simulink model "single_phase_pll_analysis"  (R2026b)
settings: Solver=ode1  StopTime=param.sim.simlength  FixedStep=param.glb_time.ts_inv
values from neighbouring files (symbols this model uses):
  param = struct()    [init_model.m]    (also in plotting_results_plls.m = evalin('base', 'param'); run_test_cases.m = param0)
undefined symbols (not defined in the file or in its folder): magnitude
libraries: discrete_time_low_pass_filter x6
settings Model: Creator=dbagn  LastModifiedBy=dbagn
settings DataIOCC: DSMLogging=off  ReturnWorkspaceOutputs=off  SaveOutput=off  SaveTime=off  SignalLogging=off
settings SimscapeCC: SimscapeUseEnergyAccounting=off

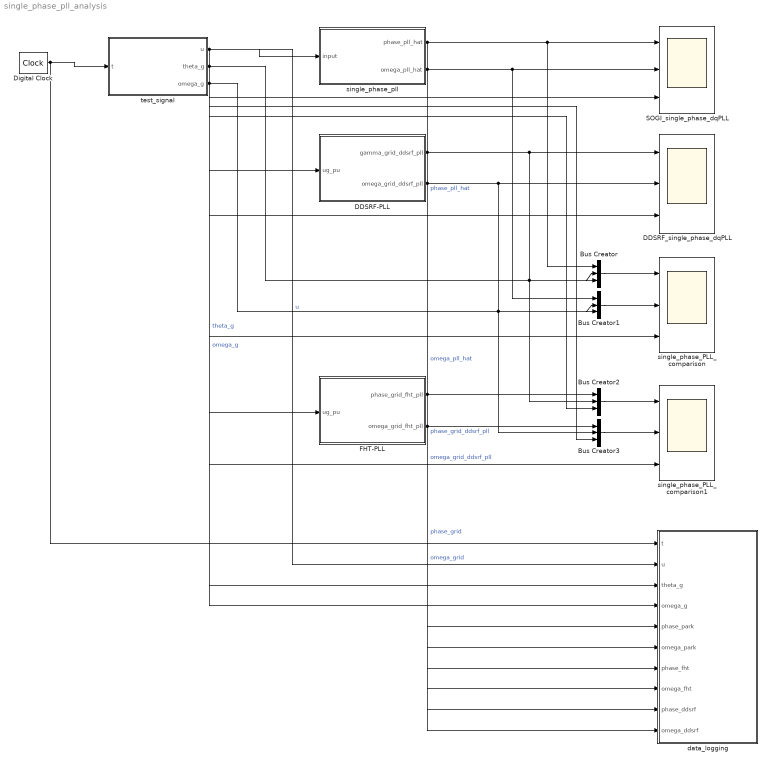
== system single_phase_pll_analysis ==
  Bus Creator{,1..3} (4 alike) : BusCreator  Inputs=3
  DDSRF-PLL : Subsystem
  DDSRF_single_phase_dqPLL : Scope  NumInputPorts=3
      settings: ActiveDisplayYMinimum=-3.9119372895053015  ActiveDisplayYMaximum=3.9180108973262389
  Digital Clock : DigitalClock  SampleTime=param.glb_time.ts_inv
  FHT-PLL : Subsystem
  SOGI_single_phase_dqPLL : Scope  NumInputPorts=3
      settings: ActiveDisplayYMinimum=-3.9194465033742367  ActiveDisplayYMaximum=3.9240760802470063  DataLoggingVariableName=ScopeData2
  data_logging : Subsystem
  single_phase_PLL_comparison : Scope  NumInputPorts=3
      settings: ActiveDisplayYMinimum=-3.9263229152471837  ActiveDisplayYMaximum=3.9266269550757258  DataLoggingVariableName=ScopeData3
  single_phase_PLL_comparison1 : Scope  NumInputPorts=3
      settings: ActiveDisplayYMinimum=-3.9176213284578751  ActiveDisplayYMaximum=3.9220307130849243  DataLoggingVariableName=ScopeData4
  single_phase_pll : Subsystem
  test_signal : MATLAB Function  TreatAsAtomicUnit=on  mask(test_signal){p=param.test}
      mask prompts: p "test signal (param.test)"
      mask help: Single-phase test voltage in pu of the nominal peak, angle theta_g and pulsation omega_g [pu] of its fundamental. p: struct of private/test_param.m (param.test).
  wires:
  DDSRF-PLL/1(gamma_grid_ddsrf_pll) -> Bus Creator2/2, Bus Creator/2, DDSRF_single_phase_dqPLL/1, data_logging/9(phase_ddsrf)  "phase_grid_ddsrf_pll"
  DDSRF-PLL/2(omega_grid_ddsrf_pll) -> Bus Creator3/2, Bus Creator1/2, DDSRF_single_phase_dqPLL/2, data_logging/10(omega_ddsrf)  "omega_grid_ddsrf_pll"
  single_phase_pll/1(phase_pll_hat) -> SOGI_single_phase_dqPLL/1, Bus Creator/1, data_logging/5(phase_park)  "phase_pll_hat"
  single_phase_pll/2(omega_pll_hat) -> Bus Creator1/1, SOGI_single_phase_dqPLL/2, data_logging/6(omega_park)  "omega_pll_hat"
  Bus Creator/1 -> single_phase_PLL_comparison/1
  Bus Creator1/1 -> single_phase_PLL_comparison/2
  Bus Creator3/1 -> single_phase_PLL_comparison1/2
  Bus Creator2/1 -> single_phase_PLL_comparison1/1
  FHT-PLL/1(phase_grid_fht_pll) -> Bus Creator2/1, data_logging/7(phase_fht)  "phase_grid"
  FHT-PLL/2(omega_grid_fht_pll) -> Bus Creator3/1, data_logging/8(omega_fht)  "omega_grid"
  Digital Clock/1 -> test_signal/1(t), data_logging/1(t)
  test_signal/1(u) -> single_phase_pll/1(input), DDSRF-PLL/1(ug_pu), FHT-PLL/1(ug_pu), SOGI_single_phase_dqPLL/3, DDSRF_single_phase_dqPLL/3, single_phase_PLL_comparison/3, single_phase_PLL_comparison1/3, data_logging/2(u)  "u"
  test_signal/2(theta_g) -> Bus Creator/3, Bus Creator2/3, data_logging/3(theta_g)  "theta_g"
  test_signal/3(omega_g) -> Bus Creator1/3, Bus Creator3/3, data_logging/4(omega_g)  "omega_g"

== system single_phase_pll_analysis/DDSRF-PLL ==
  ug_pu : Inport
  Goto Tag Visibility : GotoTagVisibility  GotoTag=Vgrid_unorm_ddsrf
  pll_stageA : Subsystem
  pll_stageB : Subsystem
  gamma_grid_ddsrf_pll : Outport
  omega_grid_ddsrf_pll : Outport  Port=2
  wires:
  pll_stageB/1(phase_grid_ddsrf_pll) -> pll_stageA/1(gamma_grid), gamma_grid_ddsrf_pll/1
  pll_stageA/2(u_grid_pos_eta) -> pll_stageB/2(u_grid_pos_eta)  "u_grid_pos_eta"
  pll_stageA/1(u_grid_pos_xi) -> pll_stageB/1(u_grid_pos_xi)  "u_grid_pos_xi"
  pll_stageB/2(omega_grid_ddsrf_pll) -> omega_grid_ddsrf_pll/1
  ug_pu/1 -> pll_stageA/2(ug_pu)

== system single_phase_pll_analysis/FHT-PLL ==
  ug_pu : Inport
  Goto Tag Visibility : GotoTagVisibility  GotoTag=Vgrid_unorm_fht
  pll_stageA : Subsystem
  pll_stageB : Subsystem
  phase_grid_fht_pll : Outport
  omega_grid_fht_pll : Outport  Port=2
  wires:
  pll_stageB/2(omega_grid_ddsrf_pll) -> omega_grid_fht_pll/1
  pll_stageA/1(u_grid_xi) -> pll_stageB/1(u_grid_pos_xi)  "u_grid_pos_xi"
  pll_stageA/2(u_grid_eta) -> pll_stageB/2(u_grid_pos_eta)  "u_grid_pos_eta"
  pll_stageB/1(phase_grid_ddsrf_pll) -> phase_grid_fht_pll/1, pll_stageA/1(gamma_grid)
  ug_pu/1 -> pll_stageA/2(ug_pu)

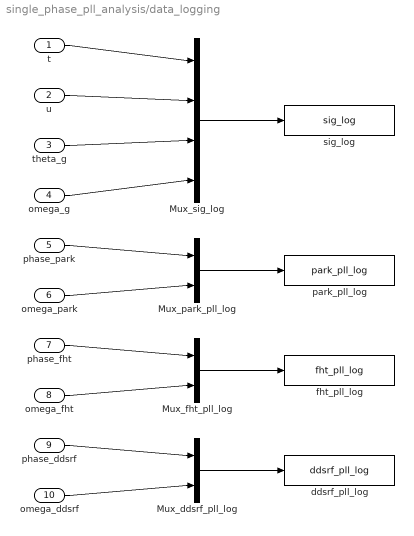
== system single_phase_pll_analysis/data_logging ==
  t : Inport
  u : Inport  Port=2
  theta_g : Inport  Port=3
  omega_g : Inport  Port=4
  phase_park : Inport  Port=5
  omega_park : Inport  Port=6
  phase_fht : Inport  Port=7
  omega_fht : Inport  Port=8
  phase_ddsrf : Inport  Port=9
  omega_ddsrf : Inport  Port=10
  Mux_ddsrf_pll_log : Mux  Inputs=2
  Mux_fht_pll_log : Mux  Inputs=2
  Mux_park_pll_log : Mux  Inputs=2
  Mux_sig_log : Mux
  ddsrf_pll_log : ToWorkspace  VariableName=ddsrf_pll_log  SampleTime=-1
      settings: MaxDataPoints=param.glb_time.Ns_afe
  fht_pll_log : ToWorkspace  VariableName=fht_pll_log  SampleTime=-1
      settings: MaxDataPoints=param.glb_time.Ns_afe
  park_pll_log : ToWorkspace  VariableName=park_pll_log  SampleTime=-1
      settings: MaxDataPoints=param.glb_time.Ns_afe
  sig_log : ToWorkspace  VariableName=sig_log  SampleTime=-1
      settings: MaxDataPoints=param.glb_time.Ns_afe
  wires:
  t/1 -> Mux_sig_log/1
  u/1 -> Mux_sig_log/2
  theta_g/1 -> Mux_sig_log/3
  omega_g/1 -> Mux_sig_log/4
  Mux_sig_log/1 -> sig_log/1
  phase_park/1 -> Mux_park_pll_log/1
  omega_park/1 -> Mux_park_pll_log/2
  Mux_park_pll_log/1 -> park_pll_log/1
  phase_fht/1 -> Mux_fht_pll_log/1
  omega_fht/1 -> Mux_fht_pll_log/2
  Mux_fht_pll_log/1 -> fht_pll_log/1
  phase_ddsrf/1 -> Mux_ddsrf_pll_log/1
  omega_ddsrf/1 -> Mux_ddsrf_pll_log/2
  Mux_ddsrf_pll_log/1 -> ddsrf_pll_log/1

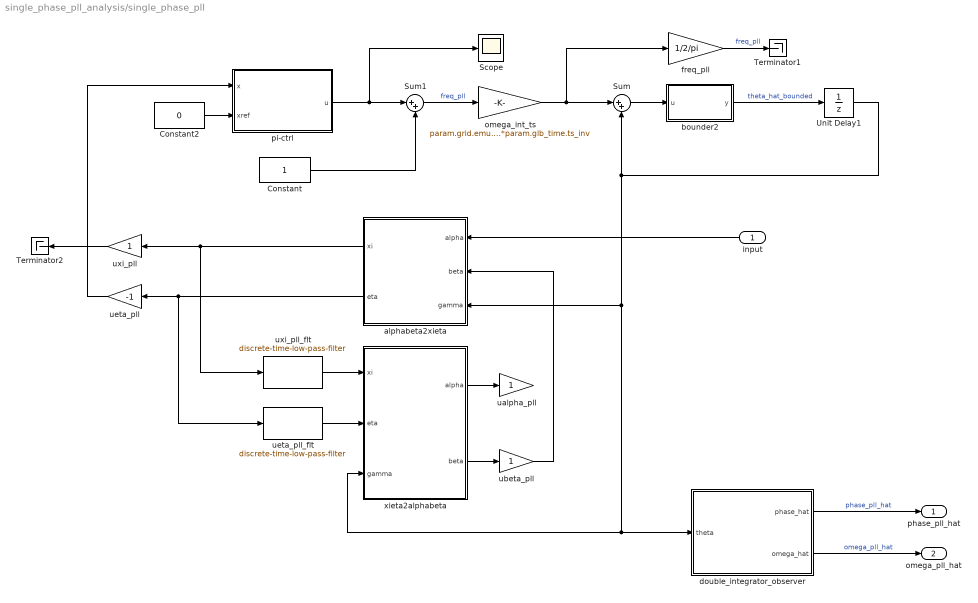
== system single_phase_pll_analysis/single_phase_pll ==
  input : Inport
  Constant : Constant
  Constant2 : Constant  Value=0
  Scope : Scope
      settings: ActiveDisplayYMinimum=-1.1813345026503461  ActiveDisplayYMaximum=0.50653477204197639
  Sum : Sum  Inputs=|++
  Sum1 : Sum  Inputs=|++
  Terminator1 : Terminator
  Terminator2 : Terminator
  Unit Delay1 : UnitDelay  SampleTime=-1
  alphabeta2xieta : MATLAB Function  TreatAsAtomicUnit=on
  bounder2 : MATLAB Function  TreatAsAtomicUnit=on
  double_integrator_observer : Subsystem
  freq_pll : Gain  Gain=1/2/pi
  omega_int_ts : Gain  Gain=param.grid.emu.omega_grid_nom*param.glb_time.ts_inv
  pi-ctrl : Subsystem  mask{kp=param.afe.pll.park.kp, ki=param.afe.pll.park.ki, ts=param.glb_time.ts_inv, sat_pos=param.afe.pll.park.sat_pos, sat_neg=param.afe.pll.park.sat_neg}
  ualpha_pll : Gain
  ubeta_pll : Gain
  ueta_pll : Gain  Gain=-1
  ueta_pll_flt : discrete_time_low_pass_filter/discrete-time-low-pass-filter  tau=param.afe.pll.park.tau  ts=param.glb_time.ts_inv
  uxi_pll : Gain
  uxi_pll_flt : discrete_time_low_pass_filter/discrete-time-low-pass-filter  tau=param.afe.pll.park.tau  ts=param.glb_time.ts_inv
  xieta2alphabeta : MATLAB Function  TreatAsAtomicUnit=on
  phase_pll_hat : Outport
  omega_pll_hat : Outport  Port=2
  wires:
  Sum/1 -> bounder2/1(u)
  alphabeta2xieta/1(xi) -> uxi_pll/1, uxi_pll_flt/1
  xieta2alphabeta/2(beta) -> ubeta_pll/1
  alphabeta2xieta/2(eta) -> ueta_pll/1, ueta_pll_flt/1
  omega_int_ts/1 -> freq_pll/1, Sum/1
  double_integrator_observer/1(phase_hat) -> phase_pll_hat/1  "phase_pll_hat"
  input/1 -> alphabeta2xieta/1(alpha)
  freq_pll/1 -> Terminator1/1  "freq_pll"
  ueta_pll_flt/1 -> xieta2alphabeta/2(eta)
  uxi_pll_flt/1 -> xieta2alphabeta/1(xi)
  ueta_pll/1 -> pi-ctrl/1(x)
  Sum1/1 -> omega_int_ts/1  "freq_pll"
  Constant2/1 -> pi-ctrl/2(xref)
  uxi_pll/1 -> Terminator2/1
  ubeta_pll/1 -> alphabeta2xieta/2(beta)
  xieta2alphabeta/1(alpha) -> ualpha_pll/1
  pi-ctrl/1(u) -> Sum1/1, Scope/1
  Constant/1 -> Sum1/2
  Unit Delay1/1 -> Sum/2, alphabeta2xieta/3(gamma), xieta2alphabeta/3(gamma), double_integrator_observer/1(theta)
  bounder2/1(y) -> Unit Delay1/1  "theta_hat_bounded"
  double_integrator_observer/2(omega_hat) -> omega_pll_hat/1  "omega_pll_hat"

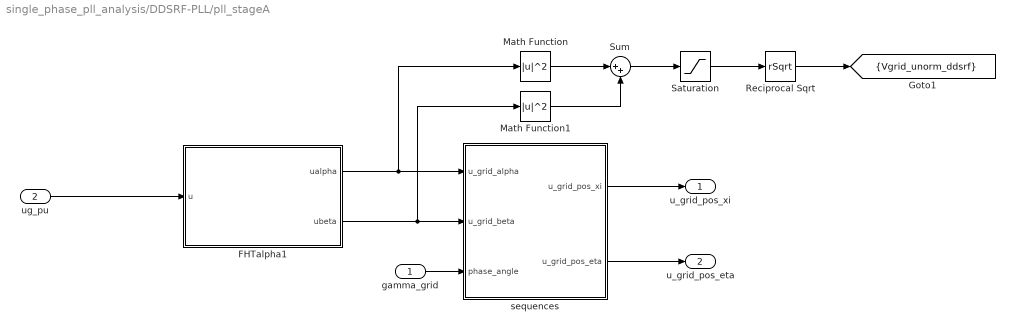
== system single_phase_pll_analysis/DDSRF-PLL/pll_stageA ==
  gamma_grid : Inport
  ug_pu : Inport  Port=2
  FHTalpha1 : Subsystem
  Math Function : Math  Operator=magnitude^2  SignedPower=on
  Math Function1 : Math  Operator=magnitude^2  SignedPower=on
  Reciprocal Sqrt : Sqrt  Operator=rSqrt
  Saturation : Saturate  UpperLimit=inf  LowerLimit=0.02
  Sum : Sum  Inputs=|++
  sequences : Subsystem
  u_grid_pos_xi : Outport  VectorParamsAs1DForOutWhenUnconnected=off
  u_grid_pos_eta : Outport  Port=2  VectorParamsAs1DForOutWhenUnconnected=off
  tag scope: Vgrid_unorm_ddsrf=scoped
  wires:
  Saturation/1 -> Reciprocal Sqrt/1
  Reciprocal Sqrt/1 -> [Vgrid_unorm_ddsrf]
  Sum/1 -> Saturation/1
  Math Function1/1 -> Sum/2
  Math Function/1 -> Sum/1
  FHTalpha1/2(ubeta) -> Math Function1/1, sequences/2(u_grid_beta)
  FHTalpha1/1(ualpha) -> Math Function/1, sequences/1(u_grid_alpha)
  sequences/1(u_grid_pos_xi) -> u_grid_pos_xi/1
  sequences/2(u_grid_pos_eta) -> u_grid_pos_eta/1
  gamma_grid/1 -> sequences/3(phase_angle)
  ug_pu/1 -> FHTalpha1/1(u)

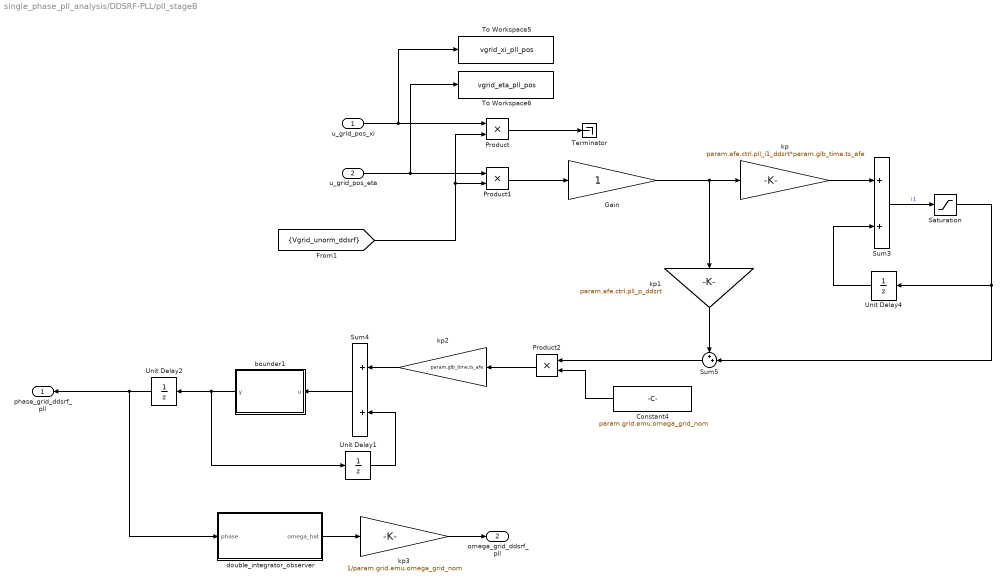
== system single_phase_pll_analysis/DDSRF-PLL/pll_stageB ==
  u_grid_pos_xi : Inport
  u_grid_pos_eta : Inport  Port=2
  Constant4 : Constant  Value=param.grid.emu.omega_grid_nom
  Gain : Gain
  Product : Product  RndMeth=Zero
  Product1 : Product  RndMeth=Zero
  Product2 : Product  RndMeth=Zero
  Saturation : Saturate  UpperLimit=1.5  LowerLimit=0.5
  Sum3 : Sum  SaturateOnIntegerOverflow=on
  Sum4 : Sum  SaturateOnIntegerOverflow=on
  Sum5 : Sum  Inputs=++|
  Terminator : Terminator
  To Workspace5 : ToWorkspace  VariableName=vgrid_xi_pll_pos  SampleTime=-1
      settings: MaxDataPoints=param.glb_time.Ns_afe
  To Workspace6 : ToWorkspace  VariableName=vgrid_eta_pll_pos  SampleTime=-1
      settings: MaxDataPoints=param.glb_time.Ns_afe
  Unit Delay1 : UnitDelay  SampleTime=-1
  Unit Delay2 : UnitDelay  SampleTime=-1
  Unit Delay4 : UnitDelay  SampleTime=-1
  bounder1 : MATLAB Function  TreatAsAtomicUnit=on
  double_integrator_observer : Subsystem
  kp : Gain  Gain=param.afe.ctrl.pll_i1_ddsrt*param.glb_time.ts_afe  SaturateOnIntegerOverflow=on  OutDataTypeStr=Inherit: Same as input  ParamDataTypeStr=Inherit: Same as input
  kp1 : Gain  Gain=param.afe.ctrl.pll_p_ddsrt  SaturateOnIntegerOverflow=on  OutDataTypeStr=Inherit: Same as input  ParamDataTypeStr=Inherit: Same as input
  kp2 : Gain  Gain=param.glb_time.ts_afe  SaturateOnIntegerOverflow=on  OutDataTypeStr=Inherit: Same as input  ParamDataTypeStr=Inherit: Same as input
  kp3 : Gain  Gain=1/param.grid.emu.omega_grid_nom  SaturateOnIntegerOverflow=on  OutDataTypeStr=Inherit: Same as input  ParamDataTypeStr=Inherit: Same as input
  phase_grid_ddsrf_pll : Outport  VectorParamsAs1DForOutWhenUnconnected=off
  omega_grid_ddsrf_pll : Outport  Port=2  VectorParamsAs1DForOutWhenUnconnected=off
  wires:
  Unit Delay2/1 -> double_integrator_observer/1(phase), phase_grid_ddsrf_pll/1
  kp1/1 -> Sum5/1
  Product2/1 -> kp2/1
  u_grid_pos_eta/1 -> Product1/1, To Workspace6/1
  u_grid_pos_xi/1 -> To Workspace5/1, Product/1
  bounder1/1(y) -> Unit Delay1/1, Unit Delay2/1
  Sum5/1 -> Product2/1
  kp/1 -> Sum3/1
  [Vgrid_unorm_ddsrf] -> Product1/2, Product/2
  Constant4/1 -> Product2/2
  kp2/1 -> Sum4/1
  Sum3/1 -> Saturation/1  "i1"
  Unit Delay1/1 -> Sum4/2
  Sum4/1 -> bounder1/1(u)
  Unit Delay4/1 -> Sum3/2
  double_integrator_observer/1(omega_hat) -> kp3/1
  Product/1 -> Terminator/1
  kp3/1 -> omega_grid_ddsrf_pll/1
  Product1/1 -> Gain/1
  Gain/1 -> kp1/1, kp/1
  Saturation/1 -> Unit Delay4/1, Sum5/2

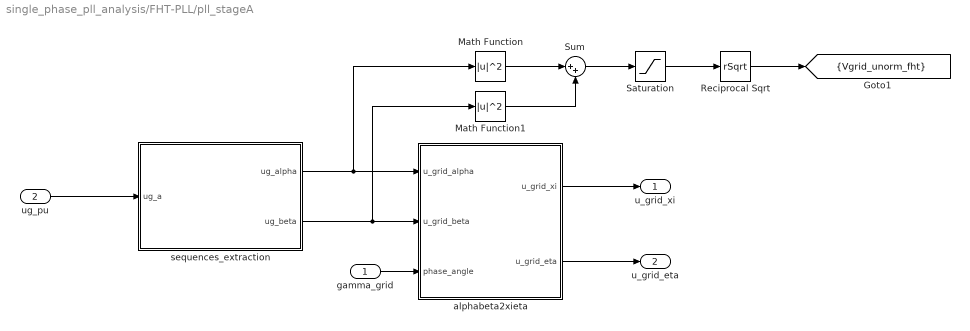
== system single_phase_pll_analysis/FHT-PLL/pll_stageA ==
  gamma_grid : Inport
  ug_pu : Inport  Port=2
  Math Function : Math  Operator=magnitude^2  SignedPower=on
  Math Function1 : Math  Operator=magnitude^2  SignedPower=on
  Reciprocal Sqrt : Sqrt  Operator=rSqrt
  Saturation : Saturate  UpperLimit=inf  LowerLimit=0.02
  Sum : Sum  Inputs=|++
  alphabeta2xieta : Subsystem
  sequences_extraction : Subsystem
  u_grid_xi : Outport  VectorParamsAs1DForOutWhenUnconnected=off
  u_grid_eta : Outport  Port=2  VectorParamsAs1DForOutWhenUnconnected=off
  tag scope: Vgrid_unorm_fht=scoped
  wires:
  gamma_grid/1 -> alphabeta2xieta/3(phase_angle)
  alphabeta2xieta/2(u_grid_eta) -> u_grid_eta/1
  alphabeta2xieta/1(u_grid_xi) -> u_grid_xi/1
  sequences_extraction/1(ug_alpha) -> Math Function/1, alphabeta2xieta/1(u_grid_alpha)
  sequences_extraction/2(ug_beta) -> Math Function1/1, alphabeta2xieta/2(u_grid_beta)
  Math Function/1 -> Sum/1
  Math Function1/1 -> Sum/2
  Sum/1 -> Saturation/1
  Reciprocal Sqrt/1 -> [Vgrid_unorm_fht]
  Saturation/1 -> Reciprocal Sqrt/1
  ug_pu/1 -> sequences_extraction/1(ug_a)

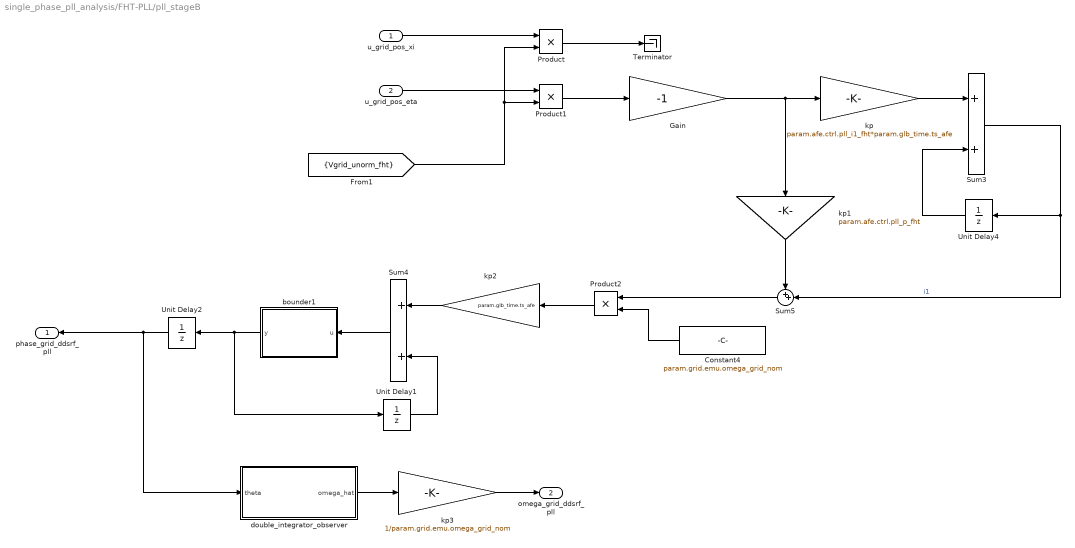
== system single_phase_pll_analysis/FHT-PLL/pll_stageB ==
  u_grid_pos_xi : Inport
  u_grid_pos_eta : Inport  Port=2
  Constant4 : Constant  Value=param.grid.emu.omega_grid_nom
  Gain : Gain  Gain=-1
  Product : Product  RndMeth=Zero
  Product1 : Product  RndMeth=Zero
  Product2 : Product  RndMeth=Zero
  Sum3 : Sum  SaturateOnIntegerOverflow=on
  Sum4 : Sum  SaturateOnIntegerOverflow=on
  Sum5 : Sum  Inputs=++|
  Terminator : Terminator
  Unit Delay1 : UnitDelay  SampleTime=-1
  Unit Delay2 : UnitDelay  SampleTime=-1
  Unit Delay4 : UnitDelay  SampleTime=-1
  bounder1 : MATLAB Function  TreatAsAtomicUnit=on
  double_integrator_observer : Subsystem
  kp : Gain  Gain=param.afe.ctrl.pll_i1_fht*param.glb_time.ts_afe  SaturateOnIntegerOverflow=on  OutDataTypeStr=Inherit: Same as input  ParamDataTypeStr=Inherit: Same as input
  kp1 : Gain  Gain=param.afe.ctrl.pll_p_fht  SaturateOnIntegerOverflow=on  OutDataTypeStr=Inherit: Same as input  ParamDataTypeStr=Inherit: Same as input
  kp2 : Gain  Gain=param.glb_time.ts_afe  SaturateOnIntegerOverflow=on  OutDataTypeStr=Inherit: Same as input  ParamDataTypeStr=Inherit: Same as input
  kp3 : Gain  Gain=1/param.grid.emu.omega_grid_nom  SaturateOnIntegerOverflow=on  OutDataTypeStr=Inherit: Same as input  ParamDataTypeStr=Inherit: Same as input
  phase_grid_ddsrf_pll : Outport  VectorParamsAs1DForOutWhenUnconnected=off
  omega_grid_ddsrf_pll : Outport  Port=2  VectorParamsAs1DForOutWhenUnconnected=off
  wires:
  Gain/1 -> kp/1, kp1/1
  Product1/1 -> Gain/1
  kp3/1 -> omega_grid_ddsrf_pll/1
  Product/1 -> Terminator/1
  double_integrator_observer/1(omega_hat) -> kp3/1
  Unit Delay4/1 -> Sum3/2
  Sum4/1 -> bounder1/1(u)
  Unit Delay1/1 -> Sum4/2
  Sum3/1 -> Sum5/2, Unit Delay4/1  "i1"
  kp2/1 -> Sum4/1
  Constant4/1 -> Product2/2
  [Vgrid_unorm_fht] -> Product/2, Product1/2
  kp/1 -> Sum3/1
  Sum5/1 -> Product2/1
  bounder1/1(y) -> Unit Delay2/1, Unit Delay1/1
  u_grid_pos_xi/1 -> Product/1
  u_grid_pos_eta/1 -> Product1/1
  Product2/1 -> kp2/1
  kp1/1 -> Sum5/1
  Unit Delay2/1 -> double_integrator_observer/1(theta), phase_grid_ddsrf_pll/1

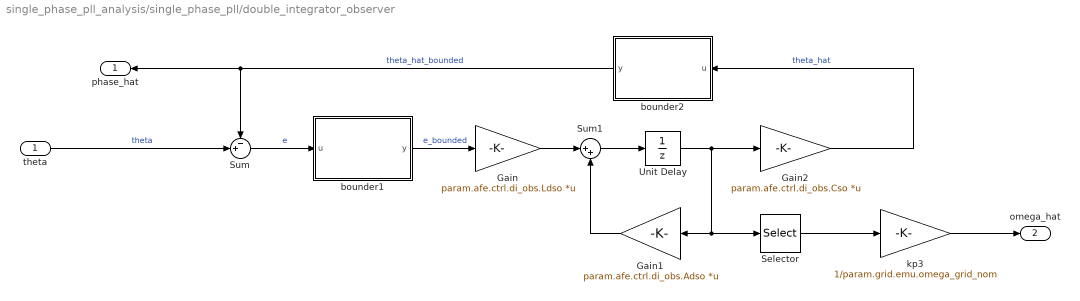
== system single_phase_pll_analysis/single_phase_pll/double_integrator_observer ==
  theta : Inport
  Gain : Gain  Gain=param.afe.ctrl.di_obs.Ldso  Multiplication=Matrix(K*u)
  Gain1 : Gain  Gain=param.afe.ctrl.di_obs.Adso  Multiplication=Matrix(K*u)
  Gain2 : Gain  Gain=param.afe.ctrl.di_obs.Cso  Multiplication=Matrix(K*u)
  Selector : Selector  InputPortWidth=2  IndexOptions=Index vector (dialog)  Indices=2  OutputSizes=1  RuntimeRangeChecks=off
  Sum : Sum  Inputs=-+|
  Sum1 : Sum  Inputs=|++
  Unit Delay : UnitDelay  SampleTime=-1
  bounder1 : MATLAB Function  TreatAsAtomicUnit=on
  bounder2 : MATLAB Function  TreatAsAtomicUnit=on
  kp3 : Gain  Gain=1/param.grid.emu.omega_grid_nom  SaturateOnIntegerOverflow=on  OutDataTypeStr=Inherit: Same as input  ParamDataTypeStr=Inherit: Same as input
  phase_hat : Outport
  omega_hat : Outport  Port=2
  wires:
  Gain/1 -> Sum1/1
  Gain2/1 -> bounder2/1(u)  "theta_hat"
  Gain1/1 -> Sum1/2
  Sum1/1 -> Unit Delay/1
  Sum/1 -> bounder1/1(u)  "e"
  Unit Delay/1 -> Selector/1, Gain1/1, Gain2/1
  theta/1 -> Sum/2  "theta"
  bounder1/1(y) -> Gain/1  "e_bounded"
  bounder2/1(y) -> phase_hat/1, Sum/1  "theta_hat_bounded"
  Selector/1 -> kp3/1
  kp3/1 -> omega_hat/1

== system single_phase_pll_analysis/single_phase_pll/pi-ctrl ==
  x : Inport
  xref : Inport  Port=2
  1/Ti : Gain  Gain=kp  SaturateOnIntegerOverflow=on  OutDataTypeStr=Inherit: Same as input  ParamDataTypeStr=Inherit: Same as input
  Saturation : Saturate  UpperLimit=sat_pos  LowerLimit=sat_neg
  Sum1 : Sum  Inputs=+++  SaturateOnIntegerOverflow=on
  Sum2 : Sum  Inputs=-+  SaturateOnIntegerOverflow=on
  Sum3 : Sum  Inputs=-+  SaturateOnIntegerOverflow=on
  Unit Delay4 : UnitDelay  SampleTime=-1
  kp : Gain  Gain=ki*ts  SaturateOnIntegerOverflow=on  OutDataTypeStr=Inherit: Same as input  ParamDataTypeStr=Inherit: Same as input
  u : Outport
  wires:
  Saturation/1 -> Sum3/2, u/1
  Unit Delay4/1 -> Sum1/3
  Sum1/1 -> Saturation/1
  Sum3/1 -> Unit Delay4/1
  1/Ti/1 -> Sum3/1, Sum1/1
  Sum2/1 -> 1/Ti/1, kp/1
  kp/1 -> Sum1/2
  x/1 -> Sum2/1
  xref/1 -> Sum2/2

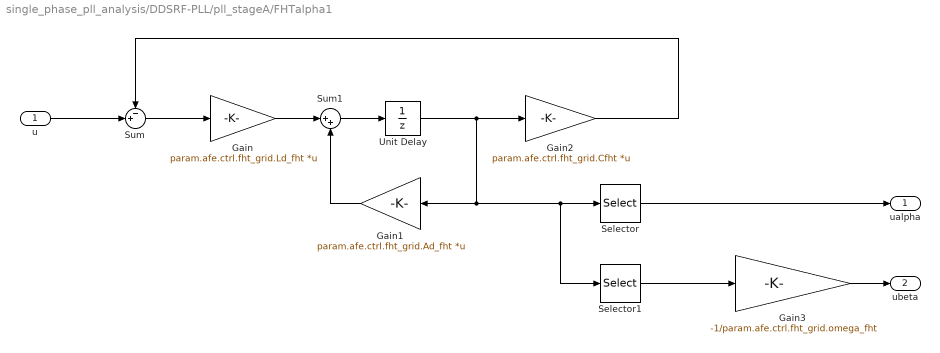
== system single_phase_pll_analysis/DDSRF-PLL/pll_stageA/FHTalpha1 ==
  u : Inport
  Gain : Gain  Gain=param.afe.ctrl.fht_grid.Ld_fht  Multiplication=Matrix(K*u)
  Gain1 : Gain  Gain=param.afe.ctrl.fht_grid.Ad_fht  Multiplication=Matrix(K*u)
  Gain2 : Gain  Gain=param.afe.ctrl.fht_grid.Cfht  Multiplication=Matrix(K*u)
  Gain3 : Gain  Gain=-1/param.afe.ctrl.fht_grid.omega_fht
  Selector : Selector  InputPortWidth=2  IndexOptions=Index vector (dialog)  Indices=1  OutputSizes=1  RuntimeRangeChecks=off
  Selector1 : Selector  InputPortWidth=2  IndexOptions=Index vector (dialog)  Indices=2  OutputSizes=1  RuntimeRangeChecks=off
  Sum : Sum  Inputs=-+|
  Sum1 : Sum  Inputs=|++
  Unit Delay : UnitDelay  SampleTime=-1
  ualpha : Outport
  ubeta : Outport  Port=2
  wires:
  u/1 -> Sum/2
  Unit Delay/1 -> Gain2/1, Selector1/1, Selector/1, Gain1/1
  Sum/1 -> Gain/1
  Sum1/1 -> Unit Delay/1
  Gain1/1 -> Sum1/2
  Gain2/1 -> Sum/1
  Selector/1 -> ualpha/1
  Gain/1 -> Sum1/1
  Selector1/1 -> Gain3/1
  Gain3/1 -> ubeta/1

== system single_phase_pll_analysis/DDSRF-PLL/pll_stageA/sequences ==
  u_grid_alpha : Inport
  u_grid_beta : Inport  Port=2
  phase_angle : Inport  Port=3
  ddsrf : Subsystem
  u_grid_pos_xi : Outport
  u_grid_pos_eta : Outport  Port=2
  wires:
  phase_angle/1 -> ddsrf/3(phase_angle)  "phase_angle"
  u_grid_beta/1 -> ddsrf/2(u_grid_beta)  "u_grid_beta"
  u_grid_alpha/1 -> ddsrf/1(u_grid_alpha)  "u_grid_alpha"
  ddsrf/1(u_grid_pos_xi) -> u_grid_pos_xi/1  "u_grid_pos_xi"
  ddsrf/2(u_grid_pos_eta) -> u_grid_pos_eta/1  "u_grid_pos_eta"

== system single_phase_pll_analysis/DDSRF-PLL/pll_stageB/double_integrator_observer ==
  phase : Inport
  Gain : Gain  Gain=param.afe.ctrl.di_obs.Ldso  Multiplication=Matrix(K*u)
  Gain1 : Gain  Gain=param.afe.ctrl.di_obs.Adso  Multiplication=Matrix(K*u)
  Gain2 : Gain  Gain=param.afe.ctrl.di_obs.Cso  Multiplication=Matrix(K*u)
  Selector : Selector  InputPortWidth=2  IndexOptions=Index vector (dialog)  Indices=2  OutputSizes=1  RuntimeRangeChecks=off
  Sum : Sum  Inputs=-+|
  Sum1 : Sum  Inputs=|++
  Unit Delay : UnitDelay  SampleTime=-1
  bounder1 : MATLAB Function  TreatAsAtomicUnit=on
  bounder2 : MATLAB Function  TreatAsAtomicUnit=on
  omega_hat : Outport
  wires:
  Gain/1 -> Sum1/1
  Selector/1 -> omega_hat/1
  Gain2/1 -> bounder2/1(u)  "theta_hat"
  Gain1/1 -> Sum1/2
  Sum1/1 -> Unit Delay/1
  Sum/1 -> bounder1/1(u)  "e"
  Unit Delay/1 -> Gain1/1, Selector/1, Gain2/1
  phase/1 -> Sum/2  "phase"
  bounder1/1(y) -> Gain/1  "e_bounded"
  bounder2/1(y) -> Sum/1  "theta_hat_bounded"

== system single_phase_pll_analysis/FHT-PLL/pll_stageA/alphabeta2xieta ==
  u_grid_alpha : Inport
  u_grid_beta : Inport  Port=2
  phase_angle : Inport  Port=3
  alphabeta2xieta : MATLAB Function  TreatAsAtomicUnit=on
  u_grid_xi : Outport
  u_grid_eta : Outport  Port=2
  wires:
  alphabeta2xieta/1(xi) -> u_grid_xi/1  "u_grid_xi"
  alphabeta2xieta/2(eta) -> u_grid_eta/1  "u_grid_eta"
  u_grid_alpha/1 -> alphabeta2xieta/1(alpha)  "u_grid_alpha"
  u_grid_beta/1 -> alphabeta2xieta/2(beta)  "u_grid_beta"
  phase_angle/1 -> alphabeta2xieta/3(gamma)  "phase_angle"

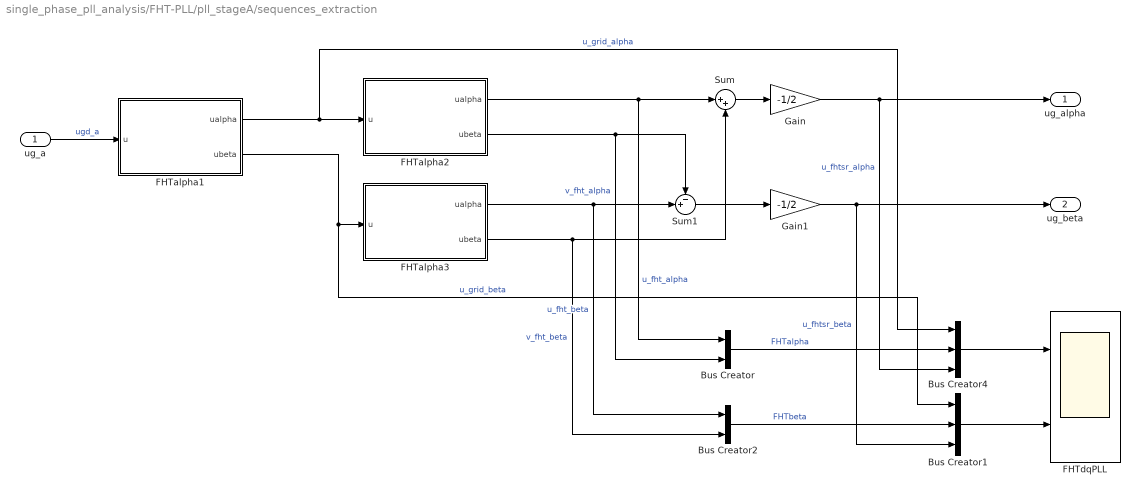
== system single_phase_pll_analysis/FHT-PLL/pll_stageA/sequences_extraction ==
  ug_a : Inport
  Bus Creator : BusCreator  Inputs=2
  Bus Creator1 : BusCreator  Inputs=3
  Bus Creator2 : BusCreator  Inputs=2
  Bus Creator4 : BusCreator  Inputs=3
  FHTalpha1 : Subsystem
  FHTalpha2 : Subsystem
  FHTalpha3 : Subsystem
  FHTdqPLL : Scope  NumInputPorts=2
      settings: ActiveDisplayYMinimum=-1.5258214459194912  ActiveDisplayYMaximum=1.5258228058860459  DataLoggingVariableName=ScopeData12
  Gain : Gain  Gain=-1/2
  Gain1 : Gain  Gain=-1/2
  Sum : Sum  Inputs=|++
  Sum1 : Sum  Inputs=-+|
  ug_alpha : Outport  VectorParamsAs1DForOutWhenUnconnected=off
  ug_beta : Outport  Port=2  VectorParamsAs1DForOutWhenUnconnected=off
  wires:
  ug_a/1 -> FHTalpha1/1(u)  "ugd_a"
  FHTalpha1/1(ualpha) -> FHTalpha2/1(u), Bus Creator4/1  "u_grid_alpha"
  FHTalpha1/2(ubeta) -> FHTalpha3/1(u), Bus Creator1/1  "u_grid_beta"
  FHTalpha2/1(ualpha) -> Bus Creator/1, Sum/1  "u_fht_alpha"
  Sum/1 -> Gain/1
  FHTalpha3/1(ualpha) -> Sum1/2, Bus Creator2/1  "u_fht_beta"
  Sum1/1 -> Gain1/1
  Gain1/1 -> Bus Creator1/3, ug_beta/1  "u_fhtsr_beta"
  Gain/1 -> Bus Creator4/3, ug_alpha/1  "u_fhtsr_alpha"
  FHTalpha3/2(ubeta) -> Sum/2, Bus Creator2/2  "v_fht_beta"
  FHTalpha2/2(ubeta) -> Sum1/1, Bus Creator/2  "v_fht_alpha"
  Bus Creator1/1 -> FHTdqPLL/2
  Bus Creator4/1 -> FHTdqPLL/1
  Bus Creator/1 -> Bus Creator4/2  "FHTalpha"
  Bus Creator2/1 -> Bus Creator1/2  "FHTbeta"

== system single_phase_pll_analysis/FHT-PLL/pll_stageB/double_integrator_observer ==
  theta : Inport
  Gain : Gain  Gain=param.afe.ctrl.di_obs.Ldso  Multiplication=Matrix(K*u)
  Gain1 : Gain  Gain=param.afe.ctrl.di_obs.Adso  Multiplication=Matrix(K*u)
  Gain2 : Gain  Gain=param.afe.ctrl.di_obs.Cso  Multiplication=Matrix(K*u)
  Selector : Selector  InputPortWidth=2  IndexOptions=Index vector (dialog)  Indices=2  OutputSizes=1  RuntimeRangeChecks=off
  Sum : Sum  Inputs=-+|
  Sum1 : Sum  Inputs=|++
  Unit Delay : UnitDelay  SampleTime=-1
  bounder1 : MATLAB Function  TreatAsAtomicUnit=on
  bounder2 : MATLAB Function  TreatAsAtomicUnit=on
  omega_hat : Outport
  wires:
  Gain/1 -> Sum1/1
  Selector/1 -> omega_hat/1
  Gain2/1 -> bounder2/1(u)  "theta_hat"
  Gain1/1 -> Sum1/2
  Sum1/1 -> Unit Delay/1
  Sum/1 -> bounder1/1(u)  "e"
  Unit Delay/1 -> Gain1/1, Selector/1, Gain2/1
  theta/1 -> Sum/2  "theta"
  bounder1/1(y) -> Gain/1
  bounder2/1(y) -> Sum/1  "theta_hat_bounded"

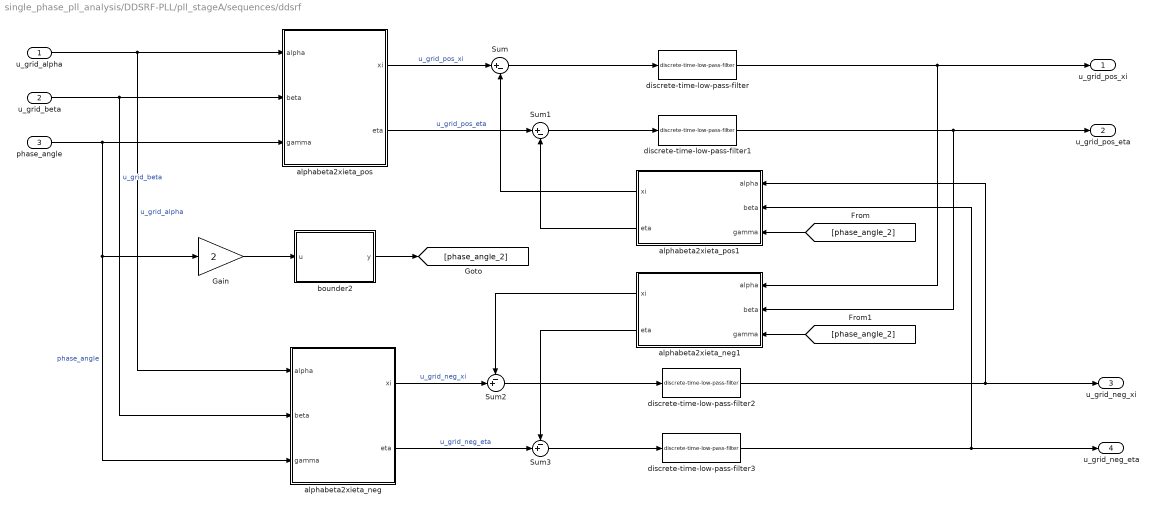
== system single_phase_pll_analysis/DDSRF-PLL/pll_stageA/sequences/ddsrf ==
  u_grid_alpha : Inport
  u_grid_beta : Inport  Port=2
  phase_angle : Inport  Port=3
  Gain : Gain  Gain=2
  Sum : Sum  Inputs=|+-
  Sum1 : Sum  Inputs=|+-
  Sum2 : Sum  Inputs=-+|
  Sum3 : Sum  Inputs=-+|
  alphabeta2xieta_neg : MATLAB Function  TreatAsAtomicUnit=on
  alphabeta2xieta_neg1 : MATLAB Function  TreatAsAtomicUnit=on
  alphabeta2xieta_pos : MATLAB Function  TreatAsAtomicUnit=on
  alphabeta2xieta_pos1 : MATLAB Function  TreatAsAtomicUnit=on
  bounder2 : MATLAB Function  TreatAsAtomicUnit=on
  discrete-time-low-pass-filter{,1..3} (4 alike) : discrete_time_low_pass_filter/discrete-time-low-pass-filter  tau=param.afe.ctrl.tau_ddsrf  ts=param.glb_time.ts_afe
  u_grid_pos_xi : Outport
  u_grid_pos_eta : Outport  Port=2
  u_grid_neg_xi : Outport  Port=3
  u_grid_neg_eta : Outport  Port=4
  wires:
  phase_angle/1 -> alphabeta2xieta_pos/3(gamma), alphabeta2xieta_neg/3(gamma), Gain/1  "phase_angle"
  u_grid_beta/1 -> alphabeta2xieta_pos/2(beta), alphabeta2xieta_neg/2(beta)  "u_grid_beta"
  u_grid_alpha/1 -> alphabeta2xieta_pos/1(alpha), alphabeta2xieta_neg/1(alpha)  "u_grid_alpha"
  alphabeta2xieta_pos/1(xi) -> Sum/1  "u_grid_pos_xi"
  Sum/1 -> discrete-time-low-pass-filter/1
  alphabeta2xieta_pos/2(eta) -> Sum1/1  "u_grid_pos_eta"
  Sum1/1 -> discrete-time-low-pass-filter1/1
  alphabeta2xieta_neg/1(xi) -> Sum2/2  "u_grid_neg_xi"
  Sum2/1 -> discrete-time-low-pass-filter2/1
  Sum3/1 -> discrete-time-low-pass-filter3/1
  alphabeta2xieta_neg/2(eta) -> Sum3/2  "u_grid_neg_eta"
  Gain/1 -> bounder2/1(u)
  discrete-time-low-pass-filter/1 -> u_grid_pos_xi/1, alphabeta2xieta_neg1/1(alpha)
  discrete-time-low-pass-filter1/1 -> u_grid_pos_eta/1, alphabeta2xieta_neg1/2(beta)
  discrete-time-low-pass-filter2/1 -> u_grid_neg_xi/1, alphabeta2xieta_pos1/1(alpha)
  discrete-time-low-pass-filter3/1 -> u_grid_neg_eta/1, alphabeta2xieta_pos1/2(beta)
  bounder2/1(y) -> [phase_angle_2]
  [phase_angle_2] -> alphabeta2xieta_pos1/3(gamma)
  [phase_angle_2] -> alphabeta2xieta_neg1/3(gamma)
  alphabeta2xieta_pos1/1(xi) -> Sum/2
  alphabeta2xieta_pos1/2(eta) -> Sum1/2
  alphabeta2xieta_neg1/1(xi) -> Sum2/1
  alphabeta2xieta_neg1/2(eta) -> Sum3/1

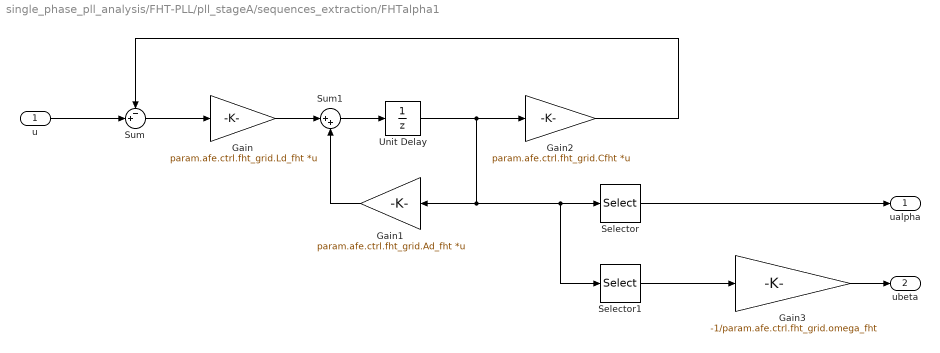
== system single_phase_pll_analysis/FHT-PLL/pll_stageA/sequences_extraction/FHTalpha1 ==
  u : Inport
  Gain : Gain  Gain=param.afe.ctrl.fht_grid.Ld_fht  Multiplication=Matrix(K*u)
  Gain1 : Gain  Gain=param.afe.ctrl.fht_grid.Ad_fht  Multiplication=Matrix(K*u)
  Gain2 : Gain  Gain=param.afe.ctrl.fht_grid.Cfht  Multiplication=Matrix(K*u)
  Gain3 : Gain  Gain=-1/param.afe.ctrl.fht_grid.omega_fht
  Selector : Selector  InputPortWidth=2  IndexOptions=Index vector (dialog)  Indices=1  OutputSizes=1  RuntimeRangeChecks=off
  Selector1 : Selector  InputPortWidth=2  IndexOptions=Index vector (dialog)  Indices=2  OutputSizes=1  RuntimeRangeChecks=off
  Sum : Sum  Inputs=-+|
  Sum1 : Sum  Inputs=|++
  Unit Delay : UnitDelay  SampleTime=-1
  ualpha : Outport
  ubeta : Outport  Port=2
  wires:
  u/1 -> Sum/2
  Unit Delay/1 -> Gain2/1, Selector1/1, Selector/1, Gain1/1
  Sum/1 -> Gain/1
  Sum1/1 -> Unit Delay/1
  Gain1/1 -> Sum1/2
  Gain2/1 -> Sum/1
  Selector/1 -> ualpha/1
  Gain/1 -> Sum1/1
  Selector1/1 -> Gain3/1
  Gain3/1 -> ubeta/1

== system single_phase_pll_analysis/FHT-PLL/pll_stageA/sequences_extraction/FHTalpha2 ==
  u : Inport
  Gain : Gain  Gain=param.afe.ctrl.fht_grid.Ld_fht  Multiplication=Matrix(K*u)
  Gain1 : Gain  Gain=param.afe.ctrl.fht_grid.Ad_fht  Multiplication=Matrix(K*u)
  Gain2 : Gain  Gain=param.afe.ctrl.fht_grid.Cfht  Multiplication=Matrix(K*u)
  Gain3 : Gain  Gain=1/param.afe.ctrl.fht_grid.omega_fht
  Selector : Selector  InputPortWidth=2  IndexOptions=Index vector (dialog)  Indices=1  OutputSizes=1  RuntimeRangeChecks=off
  Selector1 : Selector  InputPortWidth=2  IndexOptions=Index vector (dialog)  Indices=2  OutputSizes=1  RuntimeRangeChecks=off
  Sum : Sum  Inputs=-+|
  Sum1 : Sum  Inputs=|++
  Unit Delay : UnitDelay  SampleTime=-1
  ualpha : Outport
  ubeta : Outport  Port=2
  wires:
  Gain3/1 -> ubeta/1
  Selector1/1 -> Gain3/1
  Gain/1 -> Sum1/1
  Selector/1 -> ualpha/1
  Gain2/1 -> Sum/1
  Gain1/1 -> Sum1/2
  Sum1/1 -> Unit Delay/1
  Sum/1 -> Gain/1
  Unit Delay/1 -> Gain1/1, Selector/1, Selector1/1, Gain2/1
  u/1 -> Sum/2

== system single_phase_pll_analysis/FHT-PLL/pll_stageA/sequences_extraction/FHTalpha3 ==
  u : Inport
  Gain : Gain  Gain=param.afe.ctrl.fht_grid.Ld_fht  Multiplication=Matrix(K*u)
  Gain1 : Gain  Gain=param.afe.ctrl.fht_grid.Ad_fht  Multiplication=Matrix(K*u)
  Gain2 : Gain  Gain=param.afe.ctrl.fht_grid.Cfht  Multiplication=Matrix(K*u)
  Gain3 : Gain  Gain=1/param.afe.ctrl.fht_grid.omega_fht
  Selector : Selector  InputPortWidth=2  IndexOptions=Index vector (dialog)  Indices=1  OutputSizes=1  RuntimeRangeChecks=off
  Selector1 : Selector  InputPortWidth=2  IndexOptions=Index vector (dialog)  Indices=2  OutputSizes=1  RuntimeRangeChecks=off
  Sum : Sum  Inputs=-+|
  Sum1 : Sum  Inputs=|++
  Unit Delay : UnitDelay  SampleTime=-1
  ualpha : Outport
  ubeta : Outport  Port=2
  wires:
  u/1 -> Sum/2
  Unit Delay/1 -> Gain2/1, Selector1/1, Selector/1, Gain1/1
  Sum/1 -> Gain/1
  Sum1/1 -> Unit Delay/1
  Gain1/1 -> Sum1/2
  Gain2/1 -> Sum/1
  Selector/1 -> ualpha/1
  Gain/1 -> Sum1/1
  Selector1/1 -> Gain3/1
  Gain3/1 -> ubeta/1

== matlab function single_phase_pll_analysis/test_signal ==
  data: t input; u output; theta_g output; omega_g output; p parameter
function [u, theta_g, omega_g] = test_signal(t, p)
%TEST_SIGNAL  Single-phase test voltage of the PLLs, in pu of the nominal peak (p = param.test, see
%   private/test_param.m of the model).
%   phi = omega_nom t, with a frequency step to f_step omega_nom at t_fstep and a phase jump dtheta at t_jump;
%   u = A(t) (cos(phi + theta0) + sum_k harm_amp(k) sin(harm_order(k) phi + harm_phase(k))) + dc (from t_dc),
%   A(t) = a0, a_sag from t_sag, a_rec from t_rec. theta_g = phi + theta0 wrapped to (-pi, pi] is the angle of
%   the fundamental (cosine convention), omega_g its pulsation in pu of omega_nom. Inf disables an event.
w0 = p.omega_nom;
if t < p.t_fstep
    phi = w0*t;
    omega_g = 1;
else
    phi = w0*p.t_fstep + w0*p.f_step*(t - p.t_fstep);
    omega_g = p.f_step;
end
if t >= p.t_jump
    phi = phi + p.dtheta;
end
if t >= p.t_rec
    a = p.a_rec;
elseif t >= p.t_sag
    a = p.a_sag;
else
    a = p.a0;
end
u = cos(phi + p.theta0);
for k = 1:numel(p.harm_order)
    u = u + p.harm_amp(k)*sin(p.harm_order(k)*phi + p.harm_phase(k));
end
u = a*u;
if t >= p.t_dc
    u = u + p.dc;
end
theta_g = -pi + mod(phi + p.theta0 + 3*pi, 2*pi);

== matlab function single_phase_pll_analysis/FHT-PLL/pll_stageB/double_integrator_observer/bounder1 ==
  data: u input; y output
function y = bounder(u)
    
    y = -pi + mod(u+3*pi,2*pi);
    
end

== matlab function single_phase_pll_analysis/FHT-PLL/pll_stageB/double_integrator_observer/bounder2 ==
  data: u input; y output
function y = bounder(u)
    
    y = -pi + mod(u+3*pi,2*pi);
    
end

== matlab function single_phase_pll_analysis/single_phase_pll/double_integrator_observer/bounder1 ==
  data: u input; y output
function y = bounder(u)
    
    y = -pi + mod(u+3*pi,2*pi);
   
end

== matlab function single_phase_pll_analysis/single_phase_pll/double_integrator_observer/bounder2 ==
  data: u input; y output
function y = bounder(u)
    
    y = -pi + mod(u+3*pi,2*pi);
   
end

== matlab function single_phase_pll_analysis/single_phase_pll/xieta2alphabeta ==
  data: xi input; alpha output; eta input; gamma input; beta output
function [alpha,beta] = xieta2alphabeta(xi,eta,gamma)
    alpha  = xi*cos(gamma) - eta*sin(gamma);
    beta = xi*sin(gamma) + eta*cos(gamma);
end

== matlab function single_phase_pll_analysis/DDSRF-PLL/pll_stageA/sequences/ddsrf/alphabeta2xieta_neg1 ==
  data: alpha input; xi output; beta input; gamma input; eta output
function [xi,eta] = alphabeta2xieta_neg(alpha,beta,gamma)

    xi  = alpha*cos(gamma) - beta*sin(gamma);
    eta = alpha*sin(gamma) + beta*cos(gamma);

end

== matlab function single_phase_pll_analysis/DDSRF-PLL/pll_stageA/sequences/ddsrf/alphabeta2xieta_pos ==
  data: alpha input; xi output; beta input; gamma input; eta output
function [xi,eta] = alphabeta2xieta_pos(alpha,beta,gamma)

    xi  =  alpha*cos(gamma) + beta*sin(gamma);
    eta = -alpha*sin(gamma) + beta*cos(gamma);

end

== matlab function single_phase_pll_analysis/DDSRF-PLL/pll_stageA/sequences/ddsrf/alphabeta2xieta_pos1 ==
  data: alpha input; xi output; beta input; gamma input; eta output
function [xi,eta] = alphabeta2xieta_pos(alpha,beta,gamma)

    xi  =  alpha*cos(gamma) + beta*sin(gamma);
    eta = -alpha*sin(gamma) + beta*cos(gamma);

end

== matlab function single_phase_pll_analysis/DDSRF-PLL/pll_stageA/sequences/ddsrf/bounder2 ==
  data: u input; y output
function y = bounder(u)
    
    y = -pi + mod(u+3*pi,2*pi);
    % y = mod(u, 2*pi);
    
end

== matlab function single_phase_pll_analysis/DDSRF-PLL/pll_stageB/bounder1 ==
  data: u input; y output
function y = bounder(u)
    y = -pi + mod(u+3*pi,2*pi);
end

== matlab function single_phase_pll_analysis/FHT-PLL/pll_stageA/alphabeta2xieta/alphabeta2xieta ==
  data: alpha input; xi output; beta input; gamma input; eta output
function [xi,eta] = alphabeta2xieta_pos(alpha,beta,gamma)

    xi  =  (alpha*cos(gamma) + beta*sin(gamma));
    eta = (-alpha*sin(gamma) + beta*cos(gamma));

end

== matlab function single_phase_pll_analysis/single_phase_pll/alphabeta2xieta ==
  data: alpha input; xi output; beta input; gamma input; eta output
function [xi,eta] = alphabeta2xieta(alpha,beta,gamma)
    xi  =  alpha*cos(gamma) + beta*sin(gamma);
    eta = -alpha*sin(gamma) + beta*cos(gamma);
end

== matlab function single_phase_pll_analysis/single_phase_pll/bounder2 ==
  data: u input; y output
function y = bounder(u)
    
    y = -pi + mod(u+3*pi,2*pi);
   
end

== matlab function single_phase_pll_analysis/DDSRF-PLL/pll_stageA/sequences/ddsrf/alphabeta2xieta_neg ==
  data: alpha input; xi output; beta input; gamma input; eta output
function [xi,eta] = alphabeta2xieta_neg(alpha,beta,gamma)

    xi  = alpha*cos(gamma) - beta*sin(gamma);
    eta = alpha*sin(gamma) + beta*cos(gamma);

end

== matlab function single_phase_pll_analysis/DDSRF-PLL/pll_stageB/double_integrator_observer/bounder1 ==
  data: u input; y output
function y = bounder(u)
    
    y = -pi + mod(u+3*pi,2*pi);
    
end

== matlab function single_phase_pll_analysis/DDSRF-PLL/pll_stageB/double_integrator_observer/bounder2 ==
  data: u input; y output
function y = bounder(u)
    
    y = -pi + mod(u+3*pi,2*pi);
    
end

== matlab function single_phase_pll_analysis/FHT-PLL/pll_stageB/bounder1 ==
  data: u input; y output
function y = bounder(u)
    y = -pi + mod(u+3*pi,2*pi);
end
